simulink model "vtvl_sim"  (R2026a)
settings: Solver=ode45  StopTime=65  MaxStep=0.005
PreLoadFcn:
  | % Auto-load vehicle parameters
  | if exist('plant_params', 'file') == 2
  |     params = plant_params();
  | else
  |     warning('plant_params.m not found on path — params will not be loaded.');
  | end
  | 
  | % Auto-load offline ICLOCS reference trajectory
  | if exist('offline/reference_trajectory.mat', 'file') == 2
  |     load('offline/reference_trajectory.mat', 'reference');
  |     if exist('params', 'var')
  |         params.reference = reference;
  |     end
  | else
  |     warning('offline/reference_trajectory.mat not found — Mode A will not work.');
  | end
values from neighbouring files (symbols this model uses):
  reference = params.reference    [run_nominal.m]
settings Model: Creator=lucas  LastModifiedBy=lucas
settings DebuggingCC: AlgebraicLoopMsg=error  MergeDetectMultiDrivingBlocksExec=error
settings ModelReferenceCC: PropagateSignalLabelsOutOfModel=on

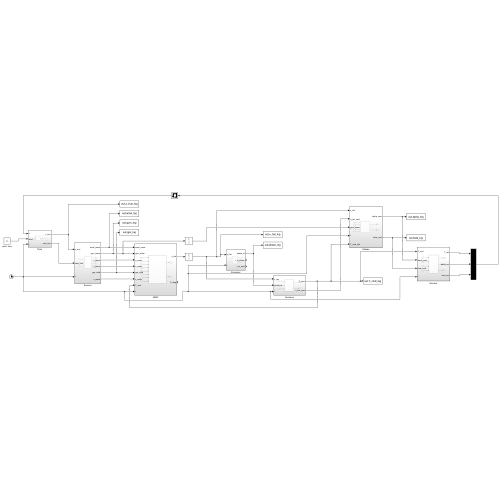
[thumbnail: Simulink's stored preview of the top-level diagram]
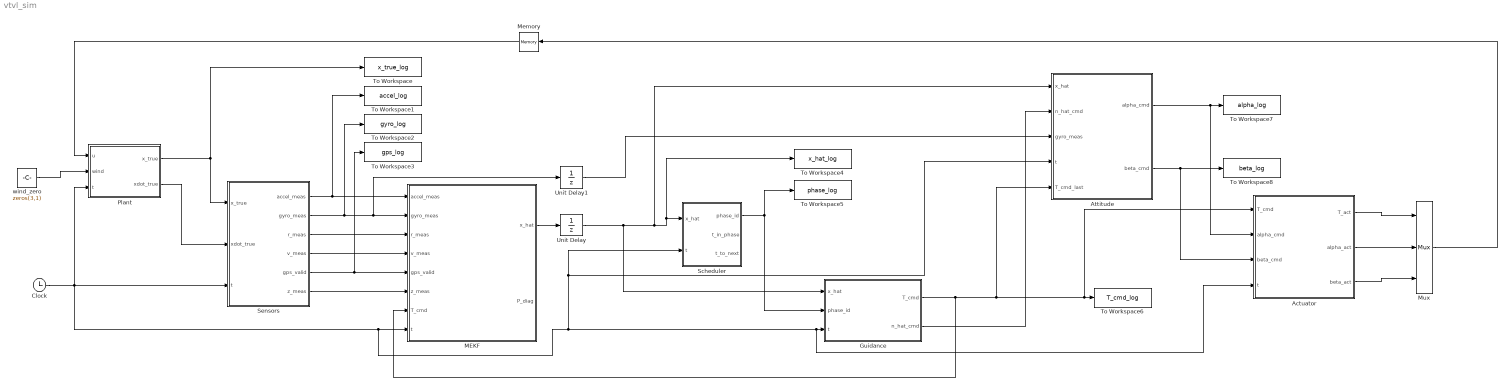
== system vtvl_sim ==
  Actuator : Subsystem
  Attitude : Subsystem
  Clock : Clock
  Guidance : Subsystem
  MEKF : Subsystem
  Memory : Memory  InitialCondition=[32; 0; 0]
  Mux : Mux  Inputs=3
  Plant : Subsystem
  Scheduler : Subsystem
  Sensors : Subsystem
  To Workspace : ToWorkspace  VariableName=x_true_log  SampleTime=0.01
      settings: Save2DSignal=2-D array (concatenate along first dimension)
  To Workspace1 : ToWorkspace  VariableName=accel_log  SampleTime=0.01
      settings: Save2DSignal=2-D array (concatenate along first dimension)
  To Workspace2 : ToWorkspace  VariableName=gyro_log  SampleTime=0.01
      settings: Save2DSignal=2-D array (concatenate along first dimension)
  To Workspace3 : ToWorkspace  VariableName=gps_log  SampleTime=0.01
      settings: Save2DSignal=2-D array (concatenate along first dimension)
  To Workspace4 : ToWorkspace  VariableName=x_hat_log  SampleTime=0.01
      settings: Save2DSignal=2-D array (concatenate along first dimension)
  To Workspace5 : ToWorkspace  VariableName=phase_log  SampleTime=0.01
      settings: Save2DSignal=2-D array (concatenate along first dimension)
  To Workspace6 : ToWorkspace  VariableName=T_cmd_log  SampleTime=0.01
      settings: Save2DSignal=2-D array (concatenate along first dimension)
  To Workspace7 : ToWorkspace  VariableName=alpha_log  SampleTime=0.005
      settings: Save2DSignal=2-D array (concatenate along first dimension)
  To Workspace8 : ToWorkspace  VariableName=beta_log  SampleTime=0.005
      settings: Save2DSignal=2-D array (concatenate along first dimension)
  Unit Delay : UnitDelay  InitialCondition=[0,0,0, 0,0,0, 1,0,0,0, 0,0,0, 0,0,0, 16.88]  SampleTime=0.005
  Unit Delay1 : UnitDelay  InitialCondition=zeros(1,3)  SampleTime=0.005
  wind_zero : Constant  Value=zeros(3,1)
  wires:
  wind_zero/1 -> Plant/2(wind)
  Plant/1(x_true) -> To Workspace/1, Sensors/1(x_true)
  Clock/1 -> Plant/3(t), Sensors/3(t), MEKF/8(t), Scheduler/2(t), Attitude/4(t), Actuator/4(t), Guidance/3(t)
  Sensors/1(accel_meas) -> To Workspace1/1, MEKF/1(accel_meas)
  Sensors/2(gyro_meas) -> To Workspace2/1, Unit Delay1/1, MEKF/2(gyro_meas)
  Sensors/5(gps_valid) -> To Workspace3/1, MEKF/5(gps_valid)
  Plant/2(xdot_true) -> Sensors/2(xdot_true)
  Sensors/3(r_meas) -> MEKF/3(r_meas)
  Sensors/4(v_meas) -> MEKF/4(v_meas)
  Sensors/6(z_meas) -> MEKF/6(z_meas)
  MEKF/1(x_hat) -> Unit Delay/1
  Scheduler/1(phase_id) -> Guidance/2(phase_id), To Workspace5/1
  Guidance/1(T_cmd) -> MEKF/7(T_cmd), Attitude/5(T_cmd_last), Actuator/1(T_cmd), To Workspace6/1
  Guidance/2(n_hat_cmd) -> Attitude/2(n_hat_cmd)
  Attitude/1(alpha_cmd) -> Actuator/2(alpha_cmd), To Workspace7/1
  Actuator/2(alpha_act) -> Mux/2
  Actuator/1(T_act) -> Mux/1
  Actuator/3(beta_act) -> Mux/3
  Mux/1 -> Memory/1
  Attitude/2(beta_cmd) -> To Workspace8/1, Actuator/3(beta_cmd)
  Unit Delay/1 -> Scheduler/1(x_hat), To Workspace4/1, Attitude/1(x_hat), Guidance/1(x_hat)
  Unit Delay1/1 -> Attitude/3(gyro_meas)
  Memory/1 -> Plant/1(u)

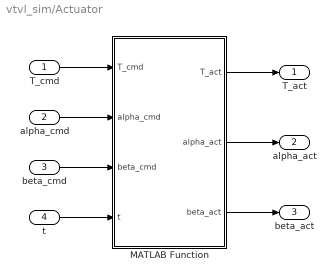
== system vtvl_sim/Actuator ==
  T_cmd : Inport
  alpha_cmd : Inport  Port=2
  beta_cmd : Inport  Port=3
  t : Inport  Port=4
  MATLAB Function : MATLAB Function  TreatAsAtomicUnit=on
  T_act : Outport
  alpha_act : Outport  Port=2
  beta_act : Outport  Port=3
  wires:
  T_cmd/1 -> MATLAB Function/1(T_cmd)
  alpha_cmd/1 -> MATLAB Function/2(alpha_cmd)
  beta_cmd/1 -> MATLAB Function/3(beta_cmd)
  t/1 -> MATLAB Function/4(t)
  MATLAB Function/1(T_act) -> T_act/1
  MATLAB Function/2(alpha_act) -> alpha_act/1
  MATLAB Function/3(beta_act) -> beta_act/1

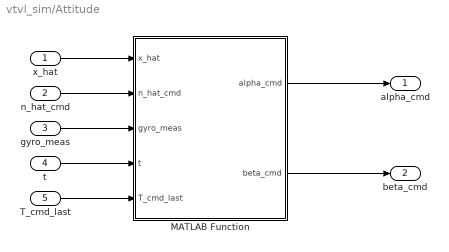
== system vtvl_sim/Attitude ==
  x_hat : Inport
  n_hat_cmd : Inport  Port=2
  gyro_meas : Inport  Port=3
  t : Inport  Port=4
  T_cmd_last : Inport  Port=5
  MATLAB Function : MATLAB Function  TreatAsAtomicUnit=on
  alpha_cmd : Outport
  beta_cmd : Outport  Port=2
  wires:
  x_hat/1 -> MATLAB Function/1(x_hat)
  n_hat_cmd/1 -> MATLAB Function/2(n_hat_cmd)
  gyro_meas/1 -> MATLAB Function/3(gyro_meas)
  t/1 -> MATLAB Function/4(t)
  MATLAB Function/2(beta_cmd) -> beta_cmd/1
  MATLAB Function/1(alpha_cmd) -> alpha_cmd/1
  T_cmd_last/1 -> MATLAB Function/5(T_cmd_last)

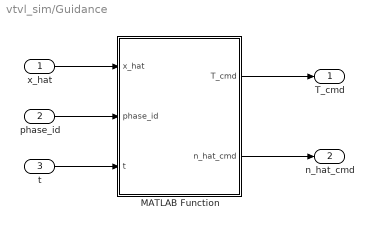
== system vtvl_sim/Guidance ==
  x_hat : Inport
  phase_id : Inport  Port=2
  t : Inport  Port=3
  MATLAB Function : MATLAB Function  TreatAsAtomicUnit=on
  T_cmd : Outport
  n_hat_cmd : Outport  Port=2
  wires:
  x_hat/1 -> MATLAB Function/1(x_hat)
  phase_id/1 -> MATLAB Function/2(phase_id)
  t/1 -> MATLAB Function/3(t)
  MATLAB Function/2(n_hat_cmd) -> n_hat_cmd/1
  MATLAB Function/1(T_cmd) -> T_cmd/1

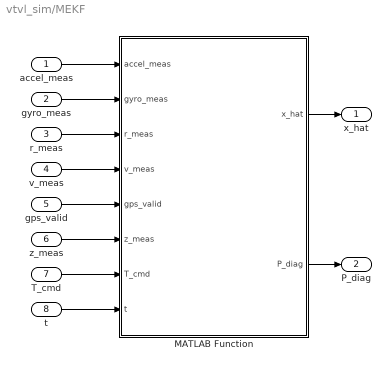
== system vtvl_sim/MEKF ==
  accel_meas : Inport
  gyro_meas : Inport  Port=2
  r_meas : Inport  Port=3
  v_meas : Inport  Port=4
  gps_valid : Inport  Port=5
  z_meas : Inport  Port=6
  T_cmd : Inport  Port=7
  t : Inport  Port=8
  MATLAB Function : MATLAB Function  TreatAsAtomicUnit=on  SystemSampleTime=0.005
  x_hat : Outport
  P_diag : Outport  Port=2
  wires:
  accel_meas/1 -> MATLAB Function/1(accel_meas)
  gyro_meas/1 -> MATLAB Function/2(gyro_meas)
  r_meas/1 -> MATLAB Function/3(r_meas)
  v_meas/1 -> MATLAB Function/4(v_meas)
  gps_valid/1 -> MATLAB Function/5(gps_valid)
  z_meas/1 -> MATLAB Function/6(z_meas)
  T_cmd/1 -> MATLAB Function/7(T_cmd)
  t/1 -> MATLAB Function/8(t)
  MATLAB Function/1(x_hat) -> x_hat/1
  MATLAB Function/2(P_diag) -> P_diag/1

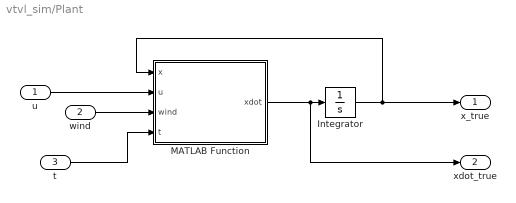
== system vtvl_sim/Plant ==
  u : Inport  OutDataTypeStr=double  PortDimensions=3
  wind : Inport  Port=2  OutDataTypeStr=double  PortDimensions=3
  t : Inport  Port=3
  Integrator : Integrator  InitialCondition=[0;0;0;0;0;0;16.88;1;0;0;0;0;0;0]
  MATLAB Function : MATLAB Function  TreatAsAtomicUnit=on
  x_true : Outport  OutDataTypeStr=double  PortDimensions=14
  xdot_true : Outport  Port=2  OutDataTypeStr=double  PortDimensions=14
  wires:
  Integrator/1 -> x_true/1, MATLAB Function/1(x)
  MATLAB Function/1(xdot) -> xdot_true/1, Integrator/1
  t/1 -> MATLAB Function/4(t)
  u/1 -> MATLAB Function/2(u)
  wind/1 -> MATLAB Function/3(wind)

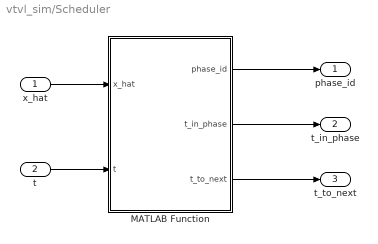
== system vtvl_sim/Scheduler ==
  x_hat : Inport
  t : Inport  Port=2
  MATLAB Function : MATLAB Function  TreatAsAtomicUnit=on
  phase_id : Outport
  t_in_phase : Outport  Port=2
  t_to_next : Outport  Port=3
  wires:
  x_hat/1 -> MATLAB Function/1(x_hat)
  t/1 -> MATLAB Function/2(t)
  MATLAB Function/3(t_to_next) -> t_to_next/1
  MATLAB Function/2(t_in_phase) -> t_in_phase/1
  MATLAB Function/1(phase_id) -> phase_id/1

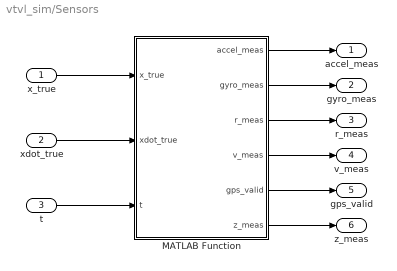
== system vtvl_sim/Sensors ==
  x_true : Inport
  xdot_true : Inport  Port=2
  t : Inport  Port=3
  MATLAB Function : MATLAB Function  TreatAsAtomicUnit=on  SystemSampleTime=0.005
  accel_meas : Outport
  gyro_meas : Outport  Port=2
  r_meas : Outport  Port=3
  v_meas : Outport  Port=4
  gps_valid : Outport  Port=5
  z_meas : Outport  Port=6
  wires:
  x_true/1 -> MATLAB Function/1(x_true)
  MATLAB Function/1(accel_meas) -> accel_meas/1
  t/1 -> MATLAB Function/3(t)
  MATLAB Function/2(gyro_meas) -> gyro_meas/1
  MATLAB Function/3(r_meas) -> r_meas/1
  MATLAB Function/4(v_meas) -> v_meas/1
  MATLAB Function/5(gps_valid) -> gps_valid/1
  MATLAB Function/6(z_meas) -> z_meas/1
  xdot_true/1 -> MATLAB Function/2(xdot_true)

== matlab function vtvl_sim/Sensors/MATLAB Function ==
  settings: updateMethod=DISCRETE  sampleTime=0.005
  data: x_true input; xdot_true input; accel_meas output; t input; gyro_meas output; r_meas output; v_meas output; gps_valid output; z_meas output
function [accel_meas, gyro_meas, r_meas, v_meas, gps_valid, z_meas] = ...
         sensors_step(x_true, xdot_true, t)
%#codegen
coder.extrinsic('sensors_wrapper');

accel_meas = zeros(1,3);
gyro_meas  = zeros(1,3);
r_meas     = zeros(1,3);
v_meas     = zeros(1,3);
gps_valid  = false;
z_meas     = 0;

% Pass xdot_true to wrapper — needed for correct IMU specific force
[accel_meas, gyro_meas, r_meas, v_meas, gps_valid, z_meas] = ...
    sensors_wrapper(x_true, xdot_true, t);
end

== matlab function vtvl_sim/Plant/MATLAB Function ==
  data: x input; u input; xdot output; wind input; t input
function xdot = plant_step(x, u, wind, t)
%#codegen

% Mark these as extrinsic — they run in MATLAB interpreter,
% not compiled. This allows evalin and complex structs.
coder.extrinsic('evalin');
coder.extrinsic('plant_dynamics');

% Declare output size explicitly BEFORE the extrinsic call.
% Required so Simulink knows xdot is 14x1 without analysing
% plant_dynamics itself.
xdot = zeros(14, 1);

% Get params from base workspace
params = evalin('base', 'params');

% Compute state derivative
xdot = plant_dynamics(x, u, t, params, wind);
end

== matlab function vtvl_sim/MEKF/MATLAB Function ==
  settings: updateMethod=DISCRETE  sampleTime=0.005
  data: accel_meas input; x_hat output; gyro_meas input; r_meas input; v_meas input; gps_valid input; z_meas input; T_cmd input; t input; P_diag output
function [x_hat, P_diag] = ekf_step(accel_meas, gyro_meas, r_meas, ...
                                      v_meas, gps_valid, z_meas, T_cmd, t)
%#codegen
coder.extrinsic('ekf_wrapper');

x_hat  = zeros(1,17);   % row vector → logs as Nx17
P_diag = zeros(1,17);

[x_hat, P_diag] = ekf_wrapper(accel_meas, gyro_meas, r_meas, v_meas, ...
                               gps_valid, z_meas, T_cmd, t);
end

== matlab function vtvl_sim/Scheduler/MATLAB Function ==
  settings: updateMethod=DISCRETE  sampleTime=0.005
  data: x_hat input; phase_id output; t input; t_in_phase output; t_to_next output
function [phase_id, t_in_phase, t_to_next] = scheduler_step(x_hat, t)
%#codegen
coder.extrinsic('scheduler_wrapper');

phase_id   = 1;
t_in_phase = 0;
t_to_next  = 0;

[phase_id, t_in_phase, t_to_next] = scheduler_wrapper(x_hat, t);
end

== matlab function vtvl_sim/Guidance/MATLAB Function ==
  settings: updateMethod=DISCRETE  sampleTime=0.5
  data: x_hat input; T_cmd output; phase_id input; t input; n_hat_cmd output
function [T_cmd, n_hat_cmd] = guidance_step(x_hat, phase_id, t)
%#codegen
coder.extrinsic('guidance_wrapper');

T_cmd     = 0;
n_hat_cmd = zeros(1,3);

[T_cmd, n_hat_cmd] = guidance_wrapper(x_hat, phase_id, t);
end

== matlab function vtvl_sim/Attitude/MATLAB Function ==
  settings: updateMethod=DISCRETE  sampleTime=0.005
  data: x_hat input; alpha_cmd output; n_hat_cmd input; gyro_meas input; t input; beta_cmd output; T_cmd_last input
function [alpha_cmd, beta_cmd] = attitude_step(x_hat, n_hat_cmd, gyro_meas, t, T_cmd_last)
%#codegen
coder.extrinsic('attitude_wrapper');

alpha_cmd = 0;
beta_cmd  = 0;

[alpha_cmd, beta_cmd] = attitude_wrapper(x_hat, n_hat_cmd, gyro_meas, t, T_cmd_last);
end

== matlab function vtvl_sim/Actuator/MATLAB Function ==
  settings: updateMethod=DISCRETE  sampleTime=0.005
  data: T_cmd input; T_act output; alpha_cmd input; beta_cmd input; t input; alpha_act output; beta_act output
function [T_act, alpha_act, beta_act] = actuator_step(T_cmd, alpha_cmd, beta_cmd, t)
%#codegen
coder.extrinsic('actuator_wrapper');

T_act     = 0;
alpha_act = 0;
beta_act  = 0;

[T_act, alpha_act, beta_act] = actuator_wrapper(T_cmd, alpha_cmd, beta_cmd, t);
end
